simulink model "MATEInductionMachineDTC"  (R2024b)
settings: Solver=FixedStepAuto  StartTime=0.0  StopTime=2.5  FixedStep=Ts  MaxStep=1e-3  RelTol=1e-3  EnableMultiTasking=on
PostLoadFcn:
  | Ts = 2e-6; MATEInductionMachineDTCInit;
InitFcn:
  | Ts = 2e-6; MATEInductionMachineDTCInit;
values from neighbouring files (symbols this model uses):
  F = 0.0106    [MATEInductionMachineDTCInit.m]
  fn = 60    [MATEInductionMachineDTCInit.m]
  H = 0.2734    [MATEInductionMachineDTCInit.m]
  Ki_wr = 3134.24    [MATEInductionMachineDTCInit.m]
  Kp_wr = 65.47    [MATEInductionMachineDTCInit.m]
  p = 2    [MATEInductionMachineDTCInit.m]
  Pn = 164e3    (= 164000)    [MATEInductionMachineDTCInit.m]
  psin = (Vn/sqrt(3)*sqrt(2)/wbase)    [MATEInductionMachineDTCInit.m]
  Tbase = Pn/(wbase/p)    (= 870.047022236)    [MATEInductionMachineDTCInit.m]
  Tsc = 1/(fsw*10)    (= 5e-05)    [MATEInductionMachineDTCInit.m]    (also in PMSMDrive_Param.m)
  Xlr = Llr*Zbase    [MATEInductionMachineDTCInit.m]
  Xls = Lls*Zbase    [MATEInductionMachineDTCInit.m]
  Xm = Lm*Zbase    [MATEInductionMachineDTCInit.m]
undefined symbols (not defined in the file or in its folder): ee
libraries: nesl_utility x15, ee_lib x11, fl_lib x9, simetranss x7, eeAsmDirectTorqueControl x2, slpidlib x2
CloseFcn:
  | clear simlog_InductionMachineDTC
  | clear logsout_InductionMachineDTC
Description:
  | Asynchronous Machine Direct Torque Control
settings Model: ModifiedByFormat=Kyle Diller  Creator=The MathWorks, Inc.  LastModifiedBy=Kyle Diller
settings SolverCC: AlgebraicLoopSolver=TrustRegion  AutoInsertRateTranBlk=on  MaxZcPerStep=1
settings DataIOCC: MaxDataPoints=510000  SaveOperatingPoint=on  SaveFormat=StructureWithTime  SaveOutput=off  ReturnWorkspaceOutputs=off  SignalLoggingName=logsout_InductionMachineDTC
settings OptimizationCC: ReuseModelBlockBuffer=off  ExpressionDepthLimit=2147483647  LifeSpan=inf
settings DebuggingCC: AlgebraicLoopMsg=error  SolverPrmCheckMsg=warning  MultiTaskRateTransMsg=warning  UnconnectedInputMsg=warning  UnconnectedOutputMsg=warning  UnconnectedLineMsg=warning  StateNameClashWarn=warning  SFUnexpectedBacktrackingDiag=warning  SFNoUnconditionalDefaultTransitionDiag=warning  SFExecutionAtInitializationDiag=none  ArithmeticOperatorsInVariantConditions=warning
settings HardwareCC: ProdBitPerPointer=32  ProdBitPerSizeT=32  ProdBitPerPtrDiffT=32  ProdLargestAtomicFloat=None  ProdIntDivRoundTo=Undefined  ProdEndianess=Unspecified  ProdWordSize=32  ProdHWDeviceType=32-bit Generic
settings ModelReferenceCC: EnableRefExpFcnMdlSchedulingChecks=on  PropagateSignalLabelsOutOfModel=off
settings SFSimCC: SimUseLocalCustomCode=off  CustomCodeUndefinedFunction=UseInterfaceOnly
settings RTWCC: RTWUseLocalCustomCode=off  GPUComputeCapability=3.5  DLArmComputeVersion=19.05
settings CodeAppCC: StateflowObjectComments=on
settings GRTTargetCC: TargetLangStandard=C89/C90 (ANSI)
settings ConfigComp: CovMetricSettings=dw  CovSaveCumulativeToWorkspaceVar=on  CovSaveSingleToWorkspaceVar=on  CovExternalEMLEnable=off  CovSFcnEnable=off
settings SimscapeCC: SimscapeLogType=all  SimscapeLogSimulationStatistics=on  SimscapeLogName=simlog_InductionMachineDTC  SimscapeLogDecimation=5  SimscapeLogDataHistory=510000

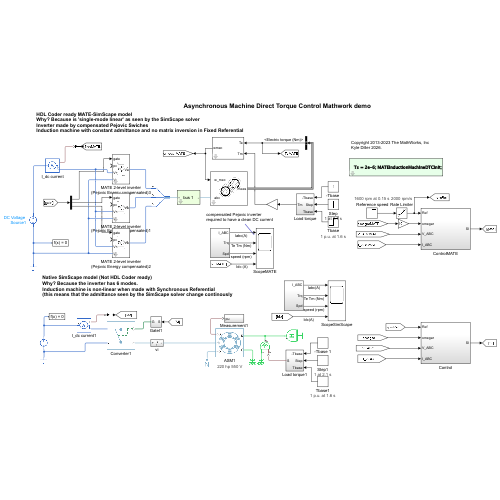
[thumbnail: Simulink's stored preview of the top-level diagram]
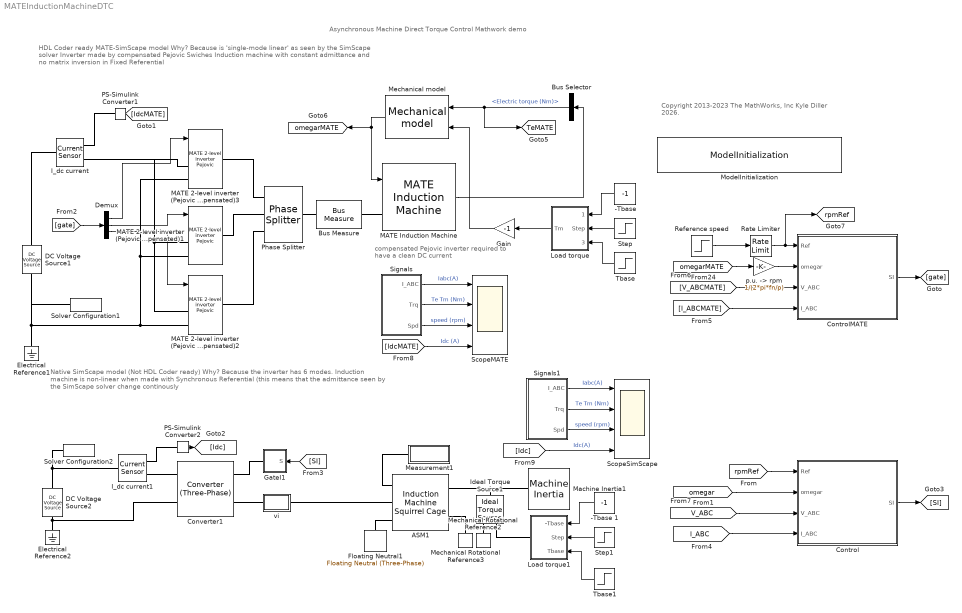
== system MATEInductionMachineDTC ==
  note: compensated Pejovic inverter
      | required to have a clean DC current
  note: Asynchronous Machine Direct Torque Control Mathwork demo
  note: Copyright 2013-2023 The MathWorks, Inc
      | Kyle Diller 2026.
  note: HDL Coder ready MATE-SimScape model
      | Why? Because is 'single-mode linear' as seen by the SimScape solver
      | Inverter made by compensated Pejovic Swiches
      | Induction machine with constant admittance and no matrix inversion in Fixed Referential
  note: Native SimScape model (Not HDL Coder ready)
      | Why? Because the inverter has 6 modes.
      | Induction machine is non-linear when made with Synchronous Referential
      | (this means that the admittance seen by the SimScape solver change continously
  " Reference speed" : Step  Time=0.15  After=1600  SampleTime=Tsc
      settings: AttributesFormatString=%<After> rpm at %<Time> s
  "-Tbase " : Constant  Value=-1  SampleTime=Ts
  -Tbase 1 : Constant  Value=-1  SampleTime=Ts
  ASM1 : ee_lib/Electromechanical/Asynchronous/Induction Machine Squirrel Cage  port_option=ee.enum.threePhasePort.composite  SRated=Pn V*A  VRated=Vn V  FRated=fn Hz  nPolePairs=p  param_unit=ee.enum.unit.si  squirrel_cage=ee.enum.squirrelcage.Single  zero_sequence=ee.enum.park.zerosequence.include  initialization_option=ee.enum.asm.initialization.fluxvariables  Rs=Rss Ohm  Xls=Xls Ohm  pu_Rs=0.0258  pu_Lls=0.0413  Rrd=Rrr Ohm  Xlrd=Xlr Ohm  pu_Rrd=0.0145  pu_Llrd=0.0424  Rrd1=0.28 Ohm  Xlrd1=0.82 Ohm  Rrd2=0.28 Ohm  Xlrd2=0.82 Ohm  pu_Rrd1=0.0290  pu_Llrd1=0.0848  pu_Rrd2=0.0290  pu_Llrd2=0.0848  Xm=Xm Ohm  pu_Lm=1.7562  X0=Xls*1000 Ohm  pu_L0=0.0413  saturation_option=0  saturation_i=[0, 4, 9, 18, 25, 34, 50, 68, 95, 120] A  saturation_v=[0, 88, 154, 198, 220, 242, 264, 286, 308, 330] V  pu_saturation_i=[0, .176, .396, .792, 1.1, 1.496, 2.2, 2.992, 4.18, 5.28]  pu_saturation_v=[0, .4, .7, .9, 1, 1.1, 1.2, 1.3, 1.4, 1.4864]  connection_option=int32(ee.enum.Connection.delta)  angular_position_specify=off  angular_position_priority=None  angular_position=0 deg  angular_position_nominal_specify=off  angular_position_nominal_value=1  angular_position_nominal_unit=deg  pu_psids_specify=off  pu_psids_priority=None  pu_psids=0  pu_psids_nominal_specify=off  pu_psids_nominal_value=1  pu_psids_nominal_unit=1  pu_psiqs_specify=off  pu_psiqs_priority=None  pu_psiqs=0  pu_psiqs_nominal_specify=off  pu_psiqs_nominal_value=1  pu_psiqs_nominal_unit=1  pu_psi0s_specify=off  pu_psi0s_priority=None  pu_psi0s=0  pu_psi0s_nominal_specify=off  pu_psi0s_nominal_value=1  pu_psi0s_nominal_unit=1  pu_psidr_specify=off  pu_psidr_priority=None  pu_psidr=0  pu_psidr_nominal_specify=off  pu_psidr_nominal_value=1  pu_psidr_nominal_unit=1  pu_psiqr_specify=off  pu_psiqr_priority=None  pu_psiqr=0  pu_psiqr_nominal_specify=off  pu_psiqr_nominal_value=1  pu_psiqr_nominal_unit=1  pu_psidr1_specify=off  pu_psidr1_priority=None  pu_psidr1=0  pu_psidr1_nominal_specify=off  pu_psidr1_nominal_value=1  pu_psidr1_nominal_unit=1  pu_psiqr1_specify=off  pu_psiqr1_priority=None  pu_psiqr1=0  pu_psiqr1_nominal_specify=off  pu_psiqr1_nominal_value=1  pu_psiqr1_nominal_unit=1  pu_psidr2_specify=off  pu_psidr2_priority=None  pu_psidr2=0  pu_psidr2_nominal_specify=off  pu_psidr2_nominal_value=1  pu_psidr2_nominal_unit=1  pu_psiqr2_specify=off  pu_psiqr2_priority=None  pu_psiqr2=0  pu_psiqr2_nominal_specify=off  pu_psiqr2_nominal_value=1  pu_psiqr2_nominal_unit=1  psids_specify=off  psids_priority=None  psids=0 Wb  psids_nominal_specify=off  psids_nominal_value=1  psids_nominal_unit=Wb  psiqs_specify=off  psiqs_priority=None  psiqs=0 Wb  psiqs_nominal_specify=off  psiqs_nominal_value=1  psiqs_nominal_unit=Wb  psi0s_specify=off  psi0s_priority=None  psi0s=0 Wb  psi0s_nominal_specify=off  psi0s_nominal_value=1  psi0s_nominal_unit=Wb  psidr_specify=off  psidr_priority=None  psidr=0 Wb  psidr_nominal_specify=off  psidr_nominal_value=1  psidr_nominal_unit=Wb  psiqr_specify=off  psiqr_priority=None  psiqr=0 Wb  psiqr_nominal_specify=off  psiqr_nominal_value=1  psiqr_nominal_unit=Wb  psidr1_specify=off  psidr1_priority=None  psidr1=0 Wb  psidr1_nominal_specify=off  psidr1_nominal_value=1  psidr1_nominal_unit=Wb  psiqr1_specify=off  psiqr1_priority=None  psiqr1=0 Wb  psiqr1_nominal_specify=off  psiqr1_nominal_value=1  psiqr1_nominal_unit=Wb  psidr2_specify=off  psidr2_priority=None  psidr2=0 Wb  psidr2_nominal_specify=off  psidr2_nominal_value=1  psidr2_nominal_unit=Wb  psiqr2_specify=off  psiqr2_priority=None  psiqr2=0 Wb  psiqr2_nominal_specify=off  psiqr2_nominal_value=1  psiqr2_nominal_unit=Wb  slip_specify=off  slip_priority=None  slip=0  slip_nominal_specify=off  slip_nominal_value=1  slip_nominal_unit=1  real_power_generated_specify=off  real_power_generated_priority=None  real_power_generated=0 W  real_power_generated_nominal_specify=off  real_power_generated_nominal_value=1  real_power_generated_nominal_unit=W  mechanical_power_consumed_specify=off  mechanical_power_consumed_priority=None  mechanical_power_consumed=0 W  mechanical_power_consumed_nominal_specify=off  mechanical_power_consumed_nominal_value=1  mechanical_power_consumed_nominal_unit=W  Tmeas=298.15 K  alpha=3.93e-3 1/K  alpha_cage=4.4e-3 1/K  stator_thermal_mass=100 J/K  rotor_thermal_mass=200 J/K  temperatureA_specify=off  temperatureA_priority=High  temperatureA=25 degC  temperatureA_nominal_specify=off  temperatureA_nominal_value=1  temperatureA_nominal_unit=degC  temperatureB_specify=off  temperatureB_priority=High  temperatureB=25 degC  temperatureB_nominal_specify=off  temperatureB_nominal_value=1  temperatureB_nominal_unit=degC  temperatureC_specify=off  temperatureC_priority=High  temperatureC=25 degC  temperatureC_nominal_specify=off  temperatureC_nominal_value=1  temperatureC_nominal_unit=degC  temperatureR_specify=off  temperatureR_priority=High  temperatureR=25 degC  temperatureR_nominal_specify=off  temperatureR_nominal_value=1  temperatureR_nominal_unit=degC
      settings: AttributesFormatString=220 hp 550 V  InternalSimscapePortConfiguration="{\"Bottom\":[],\"Left\":[{\"id\":\"R\",\"label\":\"R\",\"type\":\"foundation.mechanical.rotational.rotational\"},{\"id\":\"C\",\"label\":\"C\",\"type\":\"foundation.mechanical.rotational.rotational\"}],\"Right\":[{\"id\":\"pu_output\",\"label\":\"pu\",\"type\":\"output\"},{\"id\":\"N1\",\"label\":\"~1\",\"type\":\"foundation.electrical.three_phase\"},{\"id\":\"N2\",\"label\":\"~2\",\"type\":\"foundation.electrical.three_phase\"}],\"Top\":[]}"
  Bus Selector : BusSelector  OutputSignals=Electric torque (Nm)
  Bus Measure : simetranss/Measure/Bus Measure  VoltageMeasurement=phase-to-ground  SetLabelV=on  LabelV=V_ABCMATE  Vpu=off  VpuLL=off  CurrentMeasurement=yes  SetLabelI=on  LabelI=I_ABCMATE  Ipu=off  Pbase=100e6  Vbase=500e3  bnumber=1  dis=off
  Control : Subsystem
  ControlMATE : Subsystem
  Converter1 : ee_lib/Semiconductors & Converters/Converters/Converter (Three-Phase)  port_option=ee.enum.threePhasePort.composite  fidelity_option=ee.enum.converters.fidelity.detailed  device_type=3  showThermalPort=false  K=0  Vth=0.5 V  Vgt=1 V  Vgt_off=-1 V  Ih=1 A  Vf=0.8 V  Ron=0.001 Ohm  Rds=0.001 Ohm  Goff=1e-5 1/Ohm  Eon_scalar=22.86e-3 J  Eoff_scalar=17.14e-3 J  Eoff_natural_commutation=10e-3 J  Voff=300 V  Iout_scalar=600 A  onCurrentMeasDelay=0 s  useCurrentFromPreviousCycle=false  useVoltageFromPreviousCycle=false  diode_param=2  diode_Vf=0.8 V  diode_Ron=0.001 Ohm  diode_Goff=1e-5 1/Ohm  diode_C=50 nF  diode_iRM=-235 A  diode_iF=300 A  diode_idot=-50 A/us  diode_trr_param=1  diode_trr_factor=3  diode_trr=15 us  diode_Qrr=1.5e+3 s*uA  diode_rec_loss_model=ee.enum.diode.reverseRecoveryModel.fixed  diode_ErecVal=0 J  diode_scaleWithIandV=false  diode_ErecMat=zeros(2, 3) J  diode_TjrecVec=[298.15, 398.15] K  diode_IfrecVec=[.1, 1, 10] A  diode_IrecVal=10 A  diode_VrecVal=10 V  diode_tFilter=1 / 1000 / 100 s  thermal_network_parameterization=ee.enum.thermalNetworkTopology.external  Rth=[.08, .5] K/W  Rth_Cauer=[.08, .1, .5] K/W  Rth_Foster=[.08, .14, .22, .16] K/W  thermal_mass_parameterization=ee.enum.thermalNetwork.timeconstant  thermal_mass=[.01, .5] J/K  thermal_mass_Cauer=[.01, .1, .5] J/K  thermal_mass_Foster=[.001, .005, .05, .5] J/K  thermal_time_constant=[.001, .2] s  thermal_time_constant_Cauer=[.001, .1, .2] s  thermal_time_constant_Foster=[7e-05, .0007, .01, .08] s  thermal_mass_initial_temperatures=[25, 25] degC  thermal_mass_initial_temperatures_Cauer=[25, 25, 25] degC  junction_thermal_mass=0.01 J/K  Tvec_initial_Foster=[25, 25, 25, 25] degC  snubber_type=0  Cs=1e-7 F  Rs=0.1 Ohm  Vce_loss=[0, 150, 300] V
  DC Voltage Source1 : fl_lib/Electrical/Electrical Sources/DC Voltage Source  v0=750 V
  DC Voltage Source2 : fl_lib/Electrical/Electrical Sources/DC Voltage Source  v0=750 V
  Demux : Demux  Outputs=[2 2 2]
  Electrical Reference1 : fl_lib/Electrical/Electrical Elements/Electrical Reference
  Electrical Reference2 : fl_lib/Electrical/Electrical Elements/Electrical Reference
  Floating Neutral1 : ee_lib/Connectors & References/Floating Neutral (Three-Phase)  G_parasitic=1e-12 1/Ohm
      settings: InternalSimscapePortConfiguration="{\"Bottom\":[],\"Left\":[{\"id\":\"N\",\"label\":\"~\",\"type\":\"foundation.electrical.three_phase\"}],\"Right\":[],\"Top\":[]}"
  Gain : Gain  Gain=-1
  GateI1 : Subsystem
  I_dc current : fl_lib/Electrical/Electrical Sensors/Current Sensor
  I_dc current1 : fl_lib/Electrical/Electrical Sensors/Current Sensor
  Ideal Torque Source1 : fl_lib/Mechanical/Mechanical Sources/Ideal Torque Source
  Load torque : Subsystem
  Load torque1 : Subsystem
  MATE 2-level inverter (Pejovic Energy compensated)1 : simetranss/FPGA/MATE 2-level inverter Pejovic  Lon=1e-6  Ts=Ts
  MATE 2-level inverter (Pejovic Energy compensated)2 : simetranss/FPGA/MATE 2-level inverter Pejovic  Lon=1e-6  Ts=Ts
  MATE 2-level inverter (Pejovic Energy compensated)3 : simetranss/FPGA/MATE 2-level inverter Pejovic  Lon=1e-6  Ts=Ts
  MATE Induction Machine : simetranss/Machines/MATE Induction Machine  Rs=Rss  Lls=Xls/(2*pi*fn)  Rr=Rrr  Llr=Xlr/(2*pi*fn)  Lm=Xm/(2*pi*fn)  pp=p  Ts=Ts  disc=Backward Euler  park=Stationary
  Machine Inertia1 : ee_lib/Electromechanical/Mechanical/Machine Inertia  SRated=Pn V*A  FRated=fn Hz  nPolePairs=p  inertia_option=2  J=27548 kg*m^2  H=H s*W/V/A  damper_option=2  D=39.0509 N*m/(rad/s)  pu_D=F  initialization_option=2  fMechanical0=60 Hz  fElectrical0=0 Hz
      settings: InternalSimscapePortConfiguration="{\"Bottom\":[],\"Left\":[{\"id\":\"R\",\"label\":\"R\",\"type\":\"foundation.mechanical.rotational.rotational\"}],\"Right\":[],\"Top\":[]}"
  Measurement1 : Subsystem
  Mechanical Rotational Reference2 : fl_lib/Mechanical/Rotational Elements/Mechanical Rotational Reference
  Mechanical Rotational Reference3 : fl_lib/Mechanical/Rotational Elements/Mechanical Rotational Reference
  Mechanical model : simetranss/Machines/Mechanical model  J=2*H*Pn/((2*pi*fn/p)^2)  F=F*Pn/(2*pi*fn/p)^2  fo=0  Ts=Ts  Parameter5=|
      | Conversion from Per-Unit values
      | 
      | J=2*H*Pn/w_mec^2
      | F=D*Pn/w_mec^2
      | where:
      | J is the inertia in km.m^2 
      | H is the inertia constant in seconds.
      | F is the friction factor in N.m.s
      | D in the friction factor or damping factor in pu.
      | Pn is the nominal power of the machine
      | w_mec is the nominal mechanical rotational frequency of the machine in rad/s
  ModelInitialization : simetranss/Usefulls/ModelInitialization  InitFcnX=Ts = 2e-6; MATEInductionMachineDTCInit;  prel=off  posl=on  inif=on  strf=off
  PS-Simulink Converter1 : nesl_utility/PS-Simulink Converter  PhysicalDomain=network_engine_domain  SubClassName=ps_output  LeftPortType=input  RightPortType=output  PseudoPeriodic=off  Frequencies=[]  VectorFormat=inherit  Unit=inherit  AffineConversion=off
  PS-Simulink Converter2 : nesl_utility/PS-Simulink Converter  PhysicalDomain=network_engine_domain  SubClassName=ps_output  LeftPortType=input  RightPortType=output  PseudoPeriodic=off  Frequencies=[]  VectorFormat=inherit  Unit=inherit  AffineConversion=off
  Phase Splitter : ee_lib/Connectors & References/Phase Splitter
  Rate Limiter : RateLimiter  RisingSlewLimit=2000  FallingSlewLimit=-2000  SampleTimeMode=inherited
      settings: AttributesFormatString=%<RisingSlewLimit> rpm/s
  ScopeMATE : Scope  NumInputPorts=4
  ScopeSimScape : Scope  NumInputPorts=4
  Signals : Subsystem
  Signals1 : Subsystem
  Solver Configuration1 : nesl_utility/Solver Configuration  PhysicalDomain=network_engine_domain  SubClassName=solver  LeftPortType=input  RightPortType=generic  Tones=[]  Harmonics=[]  SimulateNoise=off  Profile=off  UseLocalSampling=off  EnableSwitchedLinearOptims=on  FrequencyDomain=off  UseCCode=off  RelTol=0.001  AbsTol=1e-06  MinStep=1e-09  ToWorkspace=off  RevertToSquareIcSolve=off  NumHomotopyIterations=100  PhasorMode=off  PhasorModeNumHarmonics=1  ConsistencySolver=NEWTON_FTOL  IndexReductionMethod=DerivativeReplacement  DoDC=off  ResidualTolerance=1e-09  ConsistencyTolSource=GLOBAL  ConsistencyAbsTol=0.001  ConsistencyRelTol=0.001  ConsistencyTolFactor=0.001  UseLocalSolver=on  LocalSolverChoice=NE_BACKWARD_EULER_ADVANCER  ResolveIndetEquations=on  FunctionEvalNumThread=1  LocalSolverSampleTime=Ts  DoFixedCost=on  MaxNonlinIter=5  MaxModeIter=2  ComputeImpulses=off  ImpulseIterations=2  LinearAlgebra=auto  LinearAlgebraNumThread=0  EquationFormulation=NE_TIME_EF  DelaysMemoryBudget=1024  AutomaticFiltering=on  FilteringTimeConstant=0.001  PartitionStorageMethod=AS_NEEDED  PartitionMemoryBudget=1024  PartitionMethod=ROBUST  MultibodyUseLocalSolver=off  MultibodyLocalSolverChoice=ODE1  MultibodyLocalSolverSampleTime=0.001
  Solver Configuration2 : nesl_utility/Solver Configuration  PhysicalDomain=network_engine_domain  SubClassName=solver  LeftPortType=input  RightPortType=generic  Tones=[]  Harmonics=[]  SimulateNoise=off  Profile=off  UseLocalSampling=off  EnableSwitchedLinearOptims=on  FrequencyDomain=off  UseCCode=off  RelTol=0.001  AbsTol=1e-06  MinStep=1e-09  ToWorkspace=off  RevertToSquareIcSolve=off  NumHomotopyIterations=100  PhasorMode=off  PhasorModeNumHarmonics=1  ConsistencySolver=NEWTON_FTOL  IndexReductionMethod=DerivativeReplacement  DoDC=off  ResidualTolerance=1e-09  ConsistencyTolSource=GLOBAL  ConsistencyAbsTol=0.001  ConsistencyRelTol=0.001  ConsistencyTolFactor=0.001  UseLocalSolver=on  LocalSolverChoice=NE_BACKWARD_EULER_ADVANCER  ResolveIndetEquations=on  FunctionEvalNumThread=1  LocalSolverSampleTime=Ts  DoFixedCost=on  MaxNonlinIter=5  MaxModeIter=2  ComputeImpulses=off  ImpulseIterations=2  LinearAlgebra=auto  LinearAlgebraNumThread=0  EquationFormulation=NE_TIME_EF  DelaysMemoryBudget=1024  AutomaticFiltering=on  FilteringTimeConstant=0.001  PartitionStorageMethod=AS_NEEDED  PartitionMemoryBudget=1024  PartitionMethod=ROBUST  MultibodyUseLocalSolver=off  MultibodyLocalSolverChoice=ODE1  MultibodyLocalSolverSampleTime=0.001
  Step : Step  Time=2.1  SampleTime=Ts
      settings: AttributesFormatString=%<After> at %<Time> s
  Step1 : Step  Time=2.1  SampleTime=Ts
      settings: AttributesFormatString=%<After> at %<Time> s
  Tbase : Step  Time=1.6  SampleTime=Ts
      settings: AttributesFormatString=%<After> p.u. at %<Time> s
  Tbase1 : Step  Time=1.6  SampleTime=Ts
      settings: AttributesFormatString=%<After> p.u. at %<Time> s
  "p.u. -> rpm" : Gain  Gain=1/(2*pi*fn/p)
  vi : Subsystem
  tag scope: TeMATE=global, omegarMATE=global, rpmRef=global
  wires:
  Signals/1(I_ABC) -> ScopeMATE/1  "Iabc(A)"
  Signals/2(Trq) -> ScopeMATE/2  "Te Tm (Nm)"
  Signals/3(Spd) -> ScopeMATE/3  "speed (rpm)"
  [omegarMATE] -> "p.u. -> rpm"/1
  [V_ABCMATE] -> ControlMATE/3(V_ABC)
  [I_ABCMATE] -> ControlMATE/4(I_ABC)
  ControlMATE/1(SI) -> [gate]
  "-Tbase "/1 -> Load torque/1(-Tbase)
  Step/1 -> Load torque/2(Step)
  Tbase/1 -> Load torque/3(Tbase)
  " Reference speed"/1 -> Rate Limiter/1
  [gate] -> Demux/1
  Demux/3 -> MATE 2-level inverter (Pejovic Energy compensated)2/1
  Demux/1 -> MATE 2-level inverter (Pejovic Energy compensated)3/1
  Demux/2 -> MATE 2-level inverter (Pejovic Energy compensated)1/1
  PS-Simulink Converter1/1 -> [IdcMATE]
  Tbase1/1 -> Load torque1/3(Tbase)
  Step1/1 -> Load torque1/2(Step)
  -Tbase 1/1 -> Load torque1/1(-Tbase)
  [SI] -> GateI1/1(S)
  Rate Limiter/1 -> [rpmRef], ControlMATE/1(Ref)
  [rpmRef] -> Control/1(Ref)
  Control/1(SI) -> [SI]
  [I_ABC] -> Control/4(I_ABC)
  [V_ABC] -> Control/3(V_ABC)
  [omegar] -> Control/2(omegar)
  Signals1/3(Spd) -> ScopeSimScape/3  "speed (rpm)"
  Signals1/2(Trq) -> ScopeSimScape/2  "Te Tm (Nm)"
  Signals1/1(I_ABC) -> ScopeSimScape/1  "Iabc(A)"
  PS-Simulink Converter2/1 -> [Idc]
  [IdcMATE] -> ScopeMATE/4  "Idc (A)"
  [Idc] -> ScopeSimScape/4  "Idc(A)"
  Load torque/1(Tm) -> Gain/1
  MATE Induction Machine/1 -> Bus Selector/1
  Mechanical model/1 -> [omegarMATE], MATE Induction Machine/1
  Bus Selector/1 -> [TeMATE], Mechanical model/1  "<Electric torque (Nm)>"
  "p.u. -> rpm"/1 -> ControlMATE/2(omegar)
  Gain/1 -> Mechanical model/2
  connections:
  MATE Induction Machine/LConn1 -- Bus Measure/RConn1
  MATE 2-level inverter (Pejovic Energy compensated)3/LConn2 -- DC Voltage Source1/RConn1 -- Solver Configuration1/RConn1 -- Electrical Reference1/LConn1 -- MATE 2-level inverter (Pejovic Energy compensated)2/LConn2 -- MATE 2-level inverter (Pejovic Energy compensated)1/LConn2
  I_dc current/RConn2 -- MATE 2-level inverter (Pejovic Energy compensated)3/LConn1 -- MATE 2-level inverter (Pejovic Energy compensated)2/LConn1 -- MATE 2-level inverter (Pejovic Energy compensated)1/LConn1
  MATE 2-level inverter (Pejovic Energy compensated)3/RConn1 -- Phase Splitter/RConn1
  MATE 2-level inverter (Pejovic Energy compensated)1/RConn1 -- Phase Splitter/RConn2
  MATE 2-level inverter (Pejovic Energy compensated)2/RConn1 -- Phase Splitter/RConn3
  I_dc current/RConn1 -- PS-Simulink Converter1/LConn1
  DC Voltage Source1/LConn1 -- I_dc current/LConn1
  DC Voltage Source2/LConn1 -- I_dc current1/LConn1 -- Solver Configuration2/RConn1
  Electrical Reference2/LConn1 -- DC Voltage Source2/RConn1 -- Converter1/RConn2
  ASM1/LConn1 -- Machine Inertia1/LConn1 -- Ideal Torque Source1/LConn1
  Mechanical Rotational Reference3/LConn1 -- ASM1/LConn2
  Floating Neutral1/LConn1 -- ASM1/RConn3
  ASM1/RConn1 -- Measurement1/RConn1
  Ideal Torque Source1/RConn2 -- Mechanical Rotational Reference2/LConn1
  vi/RConn1 -- ASM1/RConn2
  GateI1/RConn1 -- Converter1/LConn1
  vi/LConn1 -- Converter1/LConn2
  I_dc current1/RConn2 -- Converter1/RConn1
  PS-Simulink Converter2/LConn1 -- I_dc current1/RConn1
  Phase Splitter/LConn1 -- Bus Measure/LConn1
  Load torque1/RConn1 -- Ideal Torque Source1/RConn1

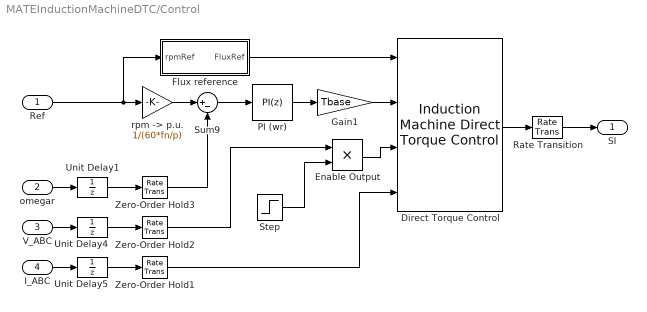
== system MATEInductionMachineDTC/Control ==
  Ref : Inport
  omegar : Inport  Port=2
  V_ABC : Inport  Port=3
  I_ABC : Inport  Port=4
  " Direct Torque Control" : eeAsmDirectTorqueControl/Induction Machine Direct Torque Control  Rs=Rss  p=p  FluxHystBand=0.2  THystBand=100  Ts=Tsc
  Enable Output : Product
  Flux reference : Subsystem
  Gain1 : Gain  Gain=Tbase
  PI (wr) : slpidlib/PID Controller  Controller=PI  Form=Parallel  TimeDomain=Discrete-time  UseExternalTs=off  SampleTime=Tsc  IntegratorMethod=Forward Euler  FilterMethod=Forward Euler  ControllerParametersSource=internal  P=Kp_wr  I=Ki_wr  UseKiTs=off  D=0  UseExternalDerivativeSource=off  N=100  UseFilter=on  TunerSelectOption=Transfer Function Based (PID Tuner App)  InitialConditionSource=internal  InitialConditionForIntegrator=0  InitialConditionForFilter=0  DifferentiatorICPrevScaledInput=0  ExternalReset=none  TrackingMode=off  Kt=1  LimitOutput=on  SatLimitsSource=internal  UpperSaturationLimit=2  LowerSaturationLimit=-2  LinearizeAsGain=on  AntiWindupMode=back-calculation  Kb=1000  LimitIntegrator=off  UpperIntegratorSaturationLimit=inf  LowerIntegratorSaturationLimit=-inf  POutMin=[]  POutMax=[]  IOutMin=[]  IOutMax=[]  DOutMin=[]  DOutMax=[]  NOutMin=[]  NOutMax=[]  SumOutMin=[]  SumOutMax=[]  SaturationOutMin=[]  SaturationOutMax=[]  PParamMin=[]  PParamMax=[]  IParamMin=[]  IParamMax=[]  DParamMin=[]  DParamMax=[]  NParamMin=[]  NParamMax=[]  KbParamMin=[]  KbParamMax=[]  KtParamMin=[]  KtParamMax=[]  KbOutMin=[]  KbOutMax=[]  KtOutMin=[]  KtOutMax=[]  IntegratorOutMin=[]  IntegratorOutMax=[]  FilterOutMin=[]  FilterOutMax=[]  SumI1OutMin=[]  SumI1OutMax=[]  SumI2OutMin=[]  SumI2OutMax=[]  SumI3OutMin=[]  SumI3OutMax=[]  SumI4OutMin=[]  SumI4OutMax=[]  SumDOutMin=[]  SumDOutMax=[]  DifferentiatorOutMin=[]  DifferentiatorOutMax=[]  FilterDiffOutCoefMin=[]  FilterDiffOutCoefMax=[]  ReciprocalOutMin=[]  ReciprocalOutMax=[]  SumDenOutMin=[]  SumDenOutMax=[]  SumNumOutMin=[]  SumNumOutMax=[]  DivideOutMin=[]  DivideOutMax=[]  UdiffTsProdOutMin=[]  UdiffTsProdOutMax=[]  NTsProdOutMin=[]  NTsProdOutMax=[]  UintegralTsProdOutMin=[]  UintegralTsProdOutMax=[]  UngainTsProdOutMin=[]  UngainTsProdOutMax=[]  ClampingZeroOutDataTypeStr=Inherit: Inherit via back propagation  ClampingZeroOutMin=[]  ClampingZeroOutMax=[]  FilterDenConstantOutDataTypeStr=Inherit: Inherit via back propagation  FilterDenConstantOutMin=[]  FilterDenConstantOutMax=[]  PCopyOutDataTypeStr=Inherit: Inherit via back propagation  PCopyOutMin=[]  PCopyOutMax=[]  NCopyOutDataTypeStr=Inherit: Inherit via back propagation  NCopyOutMin=[]  NCopyOutMax=[]  IntegratorContinuousStateAttributes=''  IntegratorStateMustResolveToSignalObject=off  IntegratorRTWStateStorageClass=Auto  FilterContinuousStateAttributes=''  FilterStateMustResolveToSignalObject=off  FilterRTWStateStorageClass=Auto  ParallelPVariant=InternalParameters  IdealPVariant=Disabled  IVariant=InternalParameters  DVariant=Disabled  IntegratorVariant=Discrete  SatVariant=Enabled  AWVariant=BackCalculation  PCopyVariant=Disabled  TRVariant=Disabled  FdbkBlocksVariant=Forward  IdealPFdbkVariant=Disabled  SatFdbkVariant=Disabled  DerivativeFilterVariant=Disabled  NVariant=Disabled  NCopyVariant=Disabled_SignalSpec  FilterICVariant=Disabled  IntegratorICVariant=InternalICs  ExternalResetVariant=Disabled  TRSumVariant=Passthrough  SumFdbkVariant=Disabled  SumVariant=Sum_PI  TsampFilterVariant=InternalTs  TsampNgainVariant=Passthrough  TsampIntegralVariant=Disabled_SignalSpec  ExternalSaturationOutDataTypeStr=Inherit: Same as second input  DerivativeSourceVariant=Disabled  PreIntVariant=InternalPreInt
  Rate Transition : RateTransition
  Step : Step  Time=0.1  SampleTime=Tsc
      settings: AttributesFormatString=%<After> at %<Time> s
  Sum9 : Sum  Inputs=|+-
  Unit Delay1 : UnitDelay  SampleTime=Ts  HasFrameUpgradeWarning=on
  Unit Delay4 : UnitDelay  SampleTime=Ts  HasFrameUpgradeWarning=on
  Unit Delay5 : UnitDelay  SampleTime=Ts  HasFrameUpgradeWarning=on
  Zero-Order Hold1 : RateTransition  OutPortSampleTime=5e-05
  Zero-Order Hold2 : RateTransition  OutPortSampleTime=5e-05
  Zero-Order Hold3 : RateTransition  OutPortSampleTime=5e-05
  "rpm -> p.u." : Gain  Gain=1/(60*fn/p)
  SI : Outport  VectorParamsAs1DForOutWhenUnconnected=off
  wires:
  Zero-Order Hold2/1 -> Enable Output/1
  Enable Output/1 -> " Direct Torque Control"/3
  Rate Transition/1 -> SI/1
  I_ABC/1 -> Unit Delay5/1
  " Direct Torque Control"/1 -> Rate Transition/1
  Unit Delay4/1 -> Zero-Order Hold2/1
  Unit Delay5/1 -> Zero-Order Hold1/1
  omegar/1 -> Unit Delay1/1
  V_ABC/1 -> Unit Delay4/1
  Ref/1 -> "rpm -> p.u."/1, Flux reference/1(rpmRef)
  Zero-Order Hold3/1 -> Sum9/2
  PI (wr)/1 -> Gain1/1
  Flux reference/1(FluxRef) -> " Direct Torque Control"/1
  Unit Delay1/1 -> Zero-Order Hold3/1
  Zero-Order Hold1/1 -> " Direct Torque Control"/4
  "rpm -> p.u."/1 -> Sum9/1
  Sum9/1 -> PI (wr)/1
  Step/1 -> Enable Output/2
  Gain1/1 -> " Direct Torque Control"/2

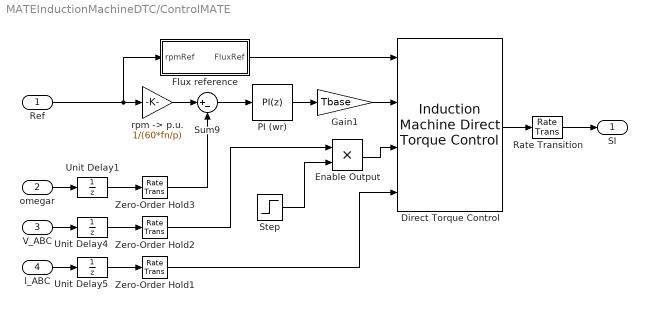
== system MATEInductionMachineDTC/ControlMATE ==
  Ref : Inport
  omegar : Inport  Port=2
  V_ABC : Inport  Port=3
  I_ABC : Inport  Port=4
  " Direct Torque Control" : eeAsmDirectTorqueControl/Induction Machine Direct Torque Control  Rs=Rss  p=p  FluxHystBand=0.2  THystBand=100  Ts=Tsc
  Enable Output : Product
  Flux reference : Subsystem
  Gain1 : Gain  Gain=Tbase
  PI (wr) : slpidlib/PID Controller  Controller=PI  Form=Parallel  TimeDomain=Discrete-time  UseExternalTs=off  SampleTime=Tsc  IntegratorMethod=Forward Euler  FilterMethod=Forward Euler  ControllerParametersSource=internal  P=Kp_wr  I=Ki_wr  UseKiTs=off  D=0  UseExternalDerivativeSource=off  N=100  UseFilter=on  TunerSelectOption=Transfer Function Based (PID Tuner App)  InitialConditionSource=internal  InitialConditionForIntegrator=0  InitialConditionForFilter=0  DifferentiatorICPrevScaledInput=0  ExternalReset=none  TrackingMode=off  Kt=1  LimitOutput=on  SatLimitsSource=internal  UpperSaturationLimit=2  LowerSaturationLimit=-2  LinearizeAsGain=on  AntiWindupMode=back-calculation  Kb=1000  LimitIntegrator=off  UpperIntegratorSaturationLimit=inf  LowerIntegratorSaturationLimit=-inf  POutMin=[]  POutMax=[]  IOutMin=[]  IOutMax=[]  DOutMin=[]  DOutMax=[]  NOutMin=[]  NOutMax=[]  SumOutMin=[]  SumOutMax=[]  SaturationOutMin=[]  SaturationOutMax=[]  PParamMin=[]  PParamMax=[]  IParamMin=[]  IParamMax=[]  DParamMin=[]  DParamMax=[]  NParamMin=[]  NParamMax=[]  KbParamMin=[]  KbParamMax=[]  KtParamMin=[]  KtParamMax=[]  KbOutMin=[]  KbOutMax=[]  KtOutMin=[]  KtOutMax=[]  IntegratorOutMin=[]  IntegratorOutMax=[]  FilterOutMin=[]  FilterOutMax=[]  SumI1OutMin=[]  SumI1OutMax=[]  SumI2OutMin=[]  SumI2OutMax=[]  SumI3OutMin=[]  SumI3OutMax=[]  SumI4OutMin=[]  SumI4OutMax=[]  SumDOutMin=[]  SumDOutMax=[]  DifferentiatorOutMin=[]  DifferentiatorOutMax=[]  FilterDiffOutCoefMin=[]  FilterDiffOutCoefMax=[]  ReciprocalOutMin=[]  ReciprocalOutMax=[]  SumDenOutMin=[]  SumDenOutMax=[]  SumNumOutMin=[]  SumNumOutMax=[]  DivideOutMin=[]  DivideOutMax=[]  UdiffTsProdOutMin=[]  UdiffTsProdOutMax=[]  NTsProdOutMin=[]  NTsProdOutMax=[]  UintegralTsProdOutMin=[]  UintegralTsProdOutMax=[]  UngainTsProdOutMin=[]  UngainTsProdOutMax=[]  ClampingZeroOutDataTypeStr=Inherit: Inherit via back propagation  ClampingZeroOutMin=[]  ClampingZeroOutMax=[]  FilterDenConstantOutDataTypeStr=Inherit: Inherit via back propagation  FilterDenConstantOutMin=[]  FilterDenConstantOutMax=[]  PCopyOutDataTypeStr=Inherit: Inherit via back propagation  PCopyOutMin=[]  PCopyOutMax=[]  NCopyOutDataTypeStr=Inherit: Inherit via back propagation  NCopyOutMin=[]  NCopyOutMax=[]  IntegratorContinuousStateAttributes=''  IntegratorStateMustResolveToSignalObject=off  IntegratorRTWStateStorageClass=Auto  FilterContinuousStateAttributes=''  FilterStateMustResolveToSignalObject=off  FilterRTWStateStorageClass=Auto  ParallelPVariant=InternalParameters  IdealPVariant=Disabled  IVariant=InternalParameters  DVariant=Disabled  IntegratorVariant=Discrete  SatVariant=Enabled  AWVariant=BackCalculation  PCopyVariant=Disabled  TRVariant=Disabled  FdbkBlocksVariant=Forward  IdealPFdbkVariant=Disabled  SatFdbkVariant=Disabled  DerivativeFilterVariant=Disabled  NVariant=Disabled  NCopyVariant=Disabled_SignalSpec  FilterICVariant=Disabled  IntegratorICVariant=InternalICs  ExternalResetVariant=Disabled  TRSumVariant=Passthrough  SumFdbkVariant=Disabled  SumVariant=Sum_PI  TsampFilterVariant=InternalTs  TsampNgainVariant=Passthrough  TsampIntegralVariant=Disabled_SignalSpec  ExternalSaturationOutDataTypeStr=Inherit: Same as second input  DerivativeSourceVariant=Disabled  PreIntVariant=InternalPreInt
  Rate Transition : RateTransition
  Step : Step  Time=0.1  SampleTime=Tsc
      settings: AttributesFormatString=%<After> at %<Time> s
  Sum9 : Sum  Inputs=|+-
  Unit Delay1 : UnitDelay  SampleTime=Ts  HasFrameUpgradeWarning=on
  Unit Delay4 : UnitDelay  SampleTime=Ts  HasFrameUpgradeWarning=on
  Unit Delay5 : UnitDelay  SampleTime=Ts  HasFrameUpgradeWarning=on
  Zero-Order Hold1 : RateTransition  OutPortSampleTime=Tsc
  Zero-Order Hold2 : RateTransition  OutPortSampleTime=Tsc
  Zero-Order Hold3 : RateTransition  OutPortSampleTime=Tsc
  "rpm -> p.u." : Gain  Gain=1/(60*fn/p)
  SI : Outport  VectorParamsAs1DForOutWhenUnconnected=off
  wires:
  Gain1/1 -> " Direct Torque Control"/2
  Step/1 -> Enable Output/2
  Sum9/1 -> PI (wr)/1
  "rpm -> p.u."/1 -> Sum9/1
  Zero-Order Hold1/1 -> " Direct Torque Control"/4
  Unit Delay1/1 -> Zero-Order Hold3/1
  Flux reference/1(FluxRef) -> " Direct Torque Control"/1
  PI (wr)/1 -> Gain1/1
  Zero-Order Hold3/1 -> Sum9/2
  Ref/1 -> Flux reference/1(rpmRef), "rpm -> p.u."/1
  V_ABC/1 -> Unit Delay4/1
  omegar/1 -> Unit Delay1/1
  Unit Delay5/1 -> Zero-Order Hold1/1
  Unit Delay4/1 -> Zero-Order Hold2/1
  " Direct Torque Control"/1 -> Rate Transition/1
  I_ABC/1 -> Unit Delay5/1
  Rate Transition/1 -> SI/1
  Enable Output/1 -> " Direct Torque Control"/3
  Zero-Order Hold2/1 -> Enable Output/1

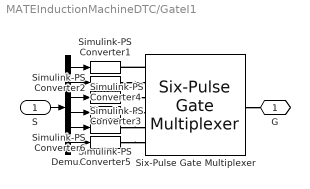
== system MATEInductionMachineDTC/GateI1 ==
  S : Inport
  Demux : Demux  Outputs=6
  Simulink-PS Converter{1..6} (6 alike) : nesl_utility/Simulink-PS Converter  PhysicalDomain=network_engine_domain  SubClassName=ps_input  LeftPortType=input  RightPortType=output  PseudoPeriodic=off  Frequencies=[]  NoiseDistribution=none  NoiseParameters=[]  Unit=1  AffineConversion=off  FilteringAndDerivatives=zero  SimscapeFilterOrder=1  InputFilterTimeConstant=0.001  UdotUserProvided=1
  Six-Pulse Gate Multiplexer : ee_lib/Semiconductors & Converters/Converters/Six-Pulse Gate Multiplexer  port_option=ee.enum.controlport.ps
  G : PMIOPort  Side=Right
  wires:
  Demux/4 -> Simulink-PS Converter4/1
  Demux/1 -> Simulink-PS Converter1/1
  Demux/2 -> Simulink-PS Converter2/1
  S/1 -> Demux/1
  Demux/5 -> Simulink-PS Converter5/1
  Demux/6 -> Simulink-PS Converter6/1
  Demux/3 -> Simulink-PS Converter3/1
  connections:
  Simulink-PS Converter4/RConn1 -- Six-Pulse Gate Multiplexer/LConn4
  Simulink-PS Converter2/RConn1 -- Six-Pulse Gate Multiplexer/LConn2
  Simulink-PS Converter3/RConn1 -- Six-Pulse Gate Multiplexer/LConn3
  Simulink-PS Converter6/RConn1 -- Six-Pulse Gate Multiplexer/LConn6
  Simulink-PS Converter5/RConn1 -- Six-Pulse Gate Multiplexer/LConn5
  Six-Pulse Gate Multiplexer/LConn1 -- Simulink-PS Converter1/RConn1
  Six-Pulse Gate Multiplexer/RConn1 -- G/RConn1

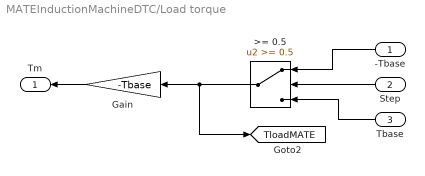
== system MATEInductionMachineDTC/Load torque ==
  -Tbase : Inport
  Step : Inport  Port=2
  Tbase : Inport  Port=3
  ">= 0.5 " : Switch  Threshold=0.5  SaturateOnIntegerOverflow=off  InputSameDT=off
  Gain : Gain  Gain=-Tbase
  Tm : Outport
  tag scope: TloadMATE=global
  wires:
  Tbase/1 -> ">= 0.5 "/3
  ">= 0.5 "/1 -> Gain/1, [TloadMATE]
  Step/1 -> ">= 0.5 "/2
  -Tbase/1 -> ">= 0.5 "/1
  Gain/1 -> Tm/1

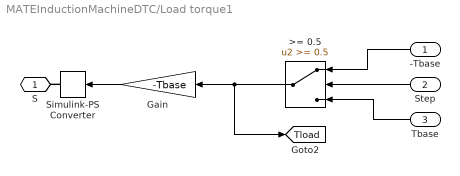
== system MATEInductionMachineDTC/Load torque1 ==
  -Tbase : Inport
  Step : Inport  Port=2
  Tbase : Inport  Port=3
  ">= 0.5 " : Switch  Threshold=0.5  SaturateOnIntegerOverflow=off  InputSameDT=off
  Gain : Gain  Gain=-Tbase
  Simulink-PS Converter : nesl_utility/Simulink-PS Converter  PhysicalDomain=network_engine_domain  SubClassName=ps_input  LeftPortType=input  RightPortType=output  PseudoPeriodic=off  Frequencies=[]  NoiseDistribution=none  NoiseParameters=[]  Unit=1  AffineConversion=off  FilteringAndDerivatives=zero  SimscapeFilterOrder=1  InputFilterTimeConstant=0.001  UdotUserProvided=1
  S : PMIOPort  Side=Right
  tag scope: Tload=global
  wires:
  -Tbase/1 -> ">= 0.5 "/1
  Step/1 -> ">= 0.5 "/2
  Gain/1 -> Simulink-PS Converter/1
  ">= 0.5 "/1 -> [Tload], Gain/1
  Tbase/1 -> ">= 0.5 "/3
  connections:
  Simulink-PS Converter/RConn1 -- S/RConn1

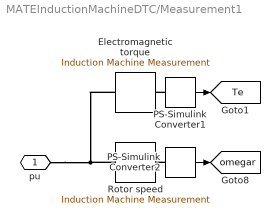
== system MATEInductionMachineDTC/Measurement1 ==
  Electromagnetic torque : ee_lib/Electromechanical/Asynchronous/Induction Machine Measurement  output_idx=1
      settings: InternalSimscapePortConfiguration="{\"Bottom\":[],\"Left\":[{\"id\":\"pu_input\",\"label\":\"pu\",\"type\":\"input\"}],\"Right\":[{\"id\":\"pu_output\",\"label\":\"o\",\"type\":\"output\"}],\"Top\":[]}"
  PS-Simulink Converter1 : nesl_utility/PS-Simulink Converter  PhysicalDomain=network_engine_domain  SubClassName=ps_output  LeftPortType=input  RightPortType=output  PseudoPeriodic=off  Frequencies=[]  VectorFormat=1-D array  Unit=1  AffineConversion=off
  PS-Simulink Converter2 : nesl_utility/PS-Simulink Converter  PhysicalDomain=network_engine_domain  SubClassName=ps_output  LeftPortType=input  RightPortType=output  PseudoPeriodic=off  Frequencies=[]  VectorFormat=1-D array  Unit=1  AffineConversion=off
  Rotor speed : ee_lib/Electromechanical/Asynchronous/Induction Machine Measurement  output_idx=2
      settings: InternalSimscapePortConfiguration="{\"Bottom\":[],\"Left\":[{\"id\":\"pu_input\",\"label\":\"pu\",\"type\":\"input\"}],\"Right\":[{\"id\":\"pu_output\",\"label\":\"o\",\"type\":\"output\"}],\"Top\":[]}"
  pu : PMIOPort  Side=Right
  tag scope: Te=global, omegar=global
  wires:
  PS-Simulink Converter1/1 -> [Te]
  PS-Simulink Converter2/1 -> [omegar]
  connections:
  Rotor speed/LConn1 -- pu/RConn1 -- Electromagnetic torque/LConn1
  PS-Simulink Converter1/LConn1 -- Electromagnetic torque/RConn1
  PS-Simulink Converter2/LConn1 -- Rotor speed/RConn1

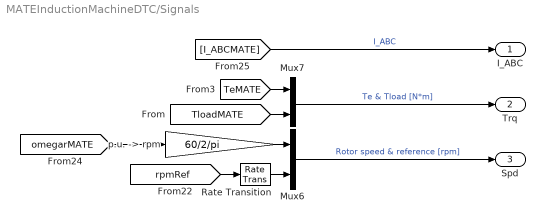
== system MATEInductionMachineDTC/Signals ==
  Mux6 : Mux  Inputs=2
  Mux7 : Mux  Inputs=2
  Rate Transition : RateTransition
  "p.u. -> rpm" : Gain  Gain=60/2/pi
  I_ABC : Outport  VectorParamsAs1DForOutWhenUnconnected=off
  Trq : Outport  Port=2  VectorParamsAs1DForOutWhenUnconnected=off
  Spd : Outport  Port=3  VectorParamsAs1DForOutWhenUnconnected=off
  wires:
  [omegarMATE] -> "p.u. -> rpm"/1
  Mux6/1 -> Spd/1  "Rotor speed & reference [rpm]"
  "p.u. -> rpm"/1 -> Mux6/1
  [rpmRef] -> Rate Transition/1
  Rate Transition/1 -> Mux6/2
  [TloadMATE] -> Mux7/2
  [I_ABCMATE] -> I_ABC/1  "I_ABC"
  [TeMATE] -> Mux7/1
  Mux7/1 -> Trq/1  "Te & Tload [N*m]"

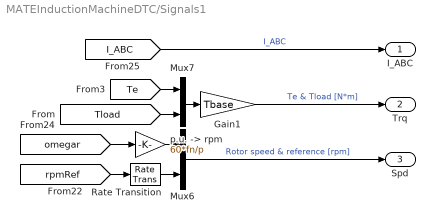
== system MATEInductionMachineDTC/Signals1 ==
  Gain1 : Gain  Gain=Tbase
  Mux6 : Mux  Inputs=2
  Mux7 : Mux  Inputs=2
  Rate Transition : RateTransition
  "p.u. -> rpm" : Gain  Gain=60*fn/p
  I_ABC : Outport  VectorParamsAs1DForOutWhenUnconnected=off
  Trq : Outport  Port=2  VectorParamsAs1DForOutWhenUnconnected=off
  Spd : Outport  Port=3  VectorParamsAs1DForOutWhenUnconnected=off
  wires:
  Gain1/1 -> Trq/1  "Te & Tload [N*m]"
  [Te] -> Mux7/1
  Mux7/1 -> Gain1/1
  [I_ABC] -> I_ABC/1  "I_ABC"
  [Tload] -> Mux7/2
  Rate Transition/1 -> Mux6/2
  [rpmRef] -> Rate Transition/1
  "p.u. -> rpm"/1 -> Mux6/1
  Mux6/1 -> Spd/1  "Rotor speed & reference [rpm]"
  [omegar] -> "p.u. -> rpm"/1

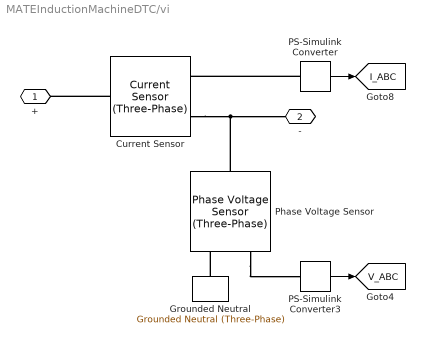
== system MATEInductionMachineDTC/vi ==
  Current Sensor : ee_lib/Sensors & Transducers/Current Sensor (Three-Phase)
  Grounded Neutral : ee_lib/Connectors & References/Grounded Neutral (Three-Phase)
  PS-Simulink Converter : nesl_utility/PS-Simulink Converter  PhysicalDomain=network_engine_domain  SubClassName=ps_output  LeftPortType=input  RightPortType=output  PseudoPeriodic=off  Frequencies=[]  VectorFormat=1-D array  Unit=A  AffineConversion=off
  PS-Simulink Converter3 : nesl_utility/PS-Simulink Converter  PhysicalDomain=network_engine_domain  SubClassName=ps_output  LeftPortType=input  RightPortType=output  PseudoPeriodic=off  Frequencies=[]  VectorFormat=1-D array  Unit=V  AffineConversion=off
  Phase Voltage Sensor : ee_lib/Sensors & Transducers/Phase Voltage Sensor (Three-Phase)
  + : PMIOPort  Side=Left
  - : PMIOPort  Port=2  Side=Right
  tag scope: I_ABC=global, V_ABC=global
  wires:
  PS-Simulink Converter3/1 -> [V_ABC]
  PS-Simulink Converter/1 -> [I_ABC]
  connections:
  Current Sensor/RConn2 -- -/RConn1 -- Phase Voltage Sensor/LConn1
  PS-Simulink Converter/LConn1 -- Current Sensor/RConn1
  Current Sensor/LConn1 -- +/RConn1
  Grounded Neutral/LConn1 -- Phase Voltage Sensor/RConn2
  Phase Voltage Sensor/RConn1 -- PS-Simulink Converter3/LConn1

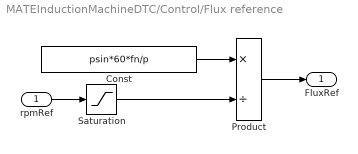
== system MATEInductionMachineDTC/Control/Flux reference ==
  rpmRef : Inport
  Const : Constant  Value=psin*60*fn/p
  Product : Product  Inputs=*/
  Saturation : Saturate  UpperLimit=inf  LowerLimit=60*fn/p
  FluxRef : Outport  VectorParamsAs1DForOutWhenUnconnected=off
  wires:
  Const/1 -> Product/1
  Saturation/1 -> Product/2
  Product/1 -> FluxRef/1
  rpmRef/1 -> Saturation/1

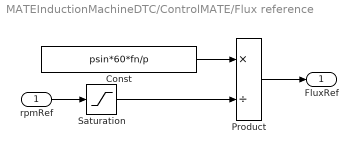
== system MATEInductionMachineDTC/ControlMATE/Flux reference ==
  rpmRef : Inport
  Const : Constant  Value=psin*60*fn/p
  Product : Product  Inputs=*/
  Saturation : Saturate  UpperLimit=inf  LowerLimit=60*fn/p
  FluxRef : Outport  VectorParamsAs1DForOutWhenUnconnected=off
  wires:
  rpmRef/1 -> Saturation/1
  Product/1 -> FluxRef/1
  Saturation/1 -> Product/2
  Const/1 -> Product/1
